simulink model "turbo_controller"  (R2025a)
settings: Solver=FixedStepAuto  StartTime=0.0  StopTime=inf  FixedStep=0.001  RelTol=1e-3
PostLoadFcn:
  | % 自动定位同目录CubeMX文件；不需要外部初始化脚本。
  | codertarget.data.setParameterValue('turbo_controller','STM32CubeMX.ProjectFile',fullfile(fileparts(get_param('turbo_controller','FileName')),'turbo_f407.ioc'));
InitFcn:
  | % 中文说明：按原控制器字段与类型创建三组接口总线；控制参数已内嵌。
  | tc_names=["EValve_Cycle" "EValve_Open" "Eblast_Cycle" "Eblast_Open" "Motor_Cycle" "Motor_Open" "EValve_Enable" "Eblast_Enable" "Motor_Enable" "SWO_Firework" "SWO_BleedAir" "EngineState" "Flag_ECUReset_Clear" "Flag_ECUReset_Save" "Flag_Reset_Enable" "Accelerator" "Nc_dem" "Nc"]; tc_types=["uint16" "uint16" "uint16" "uint16" "uint16" "uint16" "uint8" "uint8" "uint8" "uint8" "uint8" "uint8" "uint8" "uint8" "uint8" "single" "single" "single"];
  | for tc_k=1:numel(tc_names)
  |  tc_e(tc_k)=Simulink.BusElement; tc_e(tc_k).Name=char(tc_names(tc_k)); tc_e(tc_k).DataType=char(tc_types(tc_k));
  | end
  | EngineControl_Out=Simulink.Bus; EngineControl_Out.DataScope='Exported'; EngineControl_Out.Elements=tc_e;
  | clear tc_e tc_names tc_types tc_k
  | tc_names=["savedata1" "savedata2" "savedata3" "savedata4" "savedata5" "savedata6" "savedata7" "savedata8" "savedata9" "savedata10" "savedata11" "savedata12" "savedata13" "savedata14" "savedata15" "savedata16" "savedata17" "savedata18" "savedata19" "savedata20" "savedata21" "savedata22" "savedata23" "savedata24" "savedata25"]; tc_types=["single" "single" "single" "single" "single" "single" "single" "single" "single" "single" "single" "single" "single" "single" "single" "single" "single" "single" "single" "single" "single" "single" "single" "single" "single"];
  | for tc_k=1:numel(tc_names)
  |  tc_e(tc_k)=Simulink.BusElement; tc_e(tc_k).Name=char(tc_names(tc_k)); tc_e(tc_k).DataType=char(tc_types(tc_k));
  | end
  | SaveData_Out=Simulink.Bus; SaveData_Out.DataScope='Exported'; SaveData_Out.Elements=tc_e;
  | clear tc_e tc_names tc_types tc_k
  | tc_names=["senddata1" "senddata2" "senddata3" "senddata4" "senddata5" "senddata6" "senddata7" "senddata8" "senddata9" "senddata10" "senddata11" "senddata12" "senddata13" "senddata14" "senddata15" "senddata16" "senddata17" "senddata18" "senddata19" "senddata20" "senddata21" "senddata22" "senddata23" "senddata24" "senddata25" "senddata26" "senddata27" "senddata28" "senddata29"]; tc_types=["uint8" "uint8" "uint8" "uint8" "uint8" "uint8" "uint8" "uint8" "uint8" "uint8" "uint8" "uint8" "uint8" "uint8" "uint8" "uint8" "uint8" "uint8" "uint8" "uint8" "uint8" "uint8" "uint8" "uint8" "uint8" "uint8" "uint8" "uint8" "uint8"];
  | for tc_k=1:numel(tc_names)
  |  tc_e(tc_k)=Simulink.BusElement; tc_e(tc_k).Name=char(tc_names(tc_k)); tc_e(tc_k).DataType=char(tc_types(tc_k));
  | end
  | SendData_Out=Simulink.Bus; SendData_Out.DataScope='Exported'; SendData_Out.Elements=tc_e;
  | clear tc_e tc_names tc_types tc_k
  | 
  | % 以下为接口中文说明；只设置描述，不改变数值或数据类型。
  | EngineControl_Out.Description='执行控制输出（阀、电机、点火、状态及复位请求）';
  | tc_cn=["EValve_Cycle（主油阀周期计数（每计数2毫秒））" "EValve_Open（主油阀开通计数（每计数2毫秒））" "Eblast_Cycle（副油阀周期计数（每计数2毫秒））" "Eblast_Open（副油阀开通计数（每计数2毫秒））" "Motor_Cycle（起动电机周期计数）" "Motor_Open（起动电机开通计数）" "EValve_Enable（主油阀驱动使能）" "Eblast_Enable（副油阀驱动使能）" "Motor_Enable（起动电机使能）" "SWO_Firework（点火器使能（1开））" "SWO_BleedAir（引气阀使能（1开））" "EngineState（发动机状态）" "Flag_ECUReset_Clear（清除复位恢复状态请求）" "Flag_ECUReset_Save（保存复位恢复数据请求）" "Flag_Reset_Enable（处理器软件复位请求）" "Accelerator（油门／油泵给定控制量）" "Nc_dem（控制目标转速）" "Nc（发动机反馈转速（转每分））"];
  | tc_elements=EngineControl_Out.Elements;
  | for tc_k=1:numel(tc_cn)
  |  tc_elements(tc_k).Description=char(tc_cn(tc_k));
  | end
  | EngineControl_Out.Elements=tc_elements;
  | clear tc_cn tc_elements tc_k
  | SaveData_Out.Description='25项运行记录；字段含义按当前模型数据来源解释';
  | tc_cn=["savedata1（指令回显记录）" "savedata2（入口总温记录（℃））" "savedata3（电源电压记录）" "savedata4（排气温度记录（℃））" "savedata5（标定燃油压力记录）" "savedata6（副油阀占空比记录（％））" "savedata7（主油阀占空比记录（％））" "savedata8（温度修正转速记录）" "savedata9（开关输出及反馈位域）" "savedata10（物理转速记录）" "savedata11（油泵目标给定原始值）" "savedata12（起动电机占空比记录（％））" "savedata13（发动机状态码记录）" "savedata14（故障告警位域记录）" "savedata15（模型记录帧序号）" "savedata16（处理器温度记录（℃））" "savedata17（装订转速记录（沿用旧电源字段名））" "savedata18（导航高度记录）" "savedata19（飞行空速记录）" "savedata20（主阀旧记录位（恒零保留））" "savedata21（第21项保留记录（恒零））" "savedata22（保留记录项22）" "savedata23（保留记录项23）" "savedata24（保留记录项24）" "savedata25（保留记录项25）"];
  | tc_elements=SaveData_Out.Elements;
  | for tc_k=1:numel(tc_cn)
  |  tc_elements(tc_k).Description=char(tc_cn(tc_k));
  | end
  | SaveData_Out.Elements=tc_elements;
  | clear tc_cn tc_elements tc_k
  | SendData_Out.Description='29字段回传及外设命令接口；板端上位机帧只取第3至27字段';
  | tc_cn=["senddata1（回传发送允许标志（不直接上线路））" "senddata2（回传载荷长度25字节）" "senddata3（回传指令回显字节）" "senddata4（总温编码字节（℃＋80））" "senddata5（电源电压编码字节）" "senddata6（排温编码高字节）" "senddata7（排温编码低字节）" "senddata8（燃油压力编码高字节）" "senddata9（燃油压力编码低字节）" "senddata10（副油阀占空比字节（％））" "senddata11（主油阀占空比字节（％））" "senddata12（修正转速编码高字节）" "senddata13（修正转速编码低字节）" "senddata14（驱动及反馈状态位域）" "senddata15（物理转速编码高字节）" "senddata16（物理转速编码低字节）" "senddata17（油泵目标给定高字节（串口二使用））" "senddata18（油泵目标给定低字节（串口二使用））" "senddata19（起动电机占空比命令（串口一使用））" "senddata20（发动机状态码字节）" "senddata21（故障告警位域字节）" "senddata22（帧序号占位（板端另行填写））" "senddata23（处理器温度编码（℃＋50））" "senddata24（控制目标转速编码高字节）" "senddata25（控制目标转速编码低字节）" "senddata26（占位字节（板端改填实测泵速高字节））" "senddata27（占位字节（板端改填实测泵速低字节））" "senddata28（装订转速高字节（本板未发送））" "senddata29（装订转速低字节（本板未发送））"];
  | tc_elements=SendData_Out.Elements;
  | for tc_k=1:numel(tc_cn)
  |  tc_elements(tc_k).Description=char(tc_cn(tc_k));
  | end
  | SendData_Out.Elements=tc_elements;
  | clear tc_cn tc_elements tc_k
  | 
  | 
  | % FRAM模块化事务：接口类型和上电初始状态，随模型保存，无外部初始化文件。
  | clear FM_elements
  | FM_elements(1)=Simulink.BusElement;FM_elements(1).Name='phase';FM_elements(1).DataType='uint8';FM_elements(1).Dimensions=[1 1];FM_elements(1).Description='phase（当前事务阶段）';
  | FM_elements(2)=Simulink.BusElement;FM_elements(2).Name='a';FM_elements(2).DataType='uint8';FM_elements(2).Dimensions=[64 1];FM_elements(2).Description='a（启动时缓存的首区64字节）';
  | FM_elements(3)=Simulink.BusElement;FM_elements(3).Name='active';FM_elements(3).DataType='uint16';FM_elements(3).Dimensions=[1 1];FM_elements(3).Description='active（当前有效记录区地址）';
  | FM_elements(4)=Simulink.BusElement;FM_elements(4).Name='generation';FM_elements(4).DataType='uint32';FM_elements(4).Dimensions=[1 1];FM_elements(4).Description='generation（当前有效记录代号）';
  | FM_elements(5)=Simulink.BusElement;FM_elements(5).Name='record';FM_elements(5).DataType='uint8';FM_elements(5).Dimensions=[64 1];FM_elements(5).Description='record（本次冻结的待写记录）';
  | FM_elements(6)=Simulink.BusElement;FM_elements(6).Name='addr';FM_elements(6).DataType='uint16';FM_elements(6).Dimensions=[1 1];FM_elements(6).Description='addr（本次备用写入地址）';
  | FM_elements(7)=Simulink.BusElement;FM_elements(7).Name='lastSave';FM_elements(7).DataType='single';FM_elements(7).Dimensions=[1 1];FM_elements(7).Description='lastSave（上次开始保存的秒数）';
  | FM_elements(8)=Simulink.BusElement;FM_elements(8).Name='lastState';FM_elements(8).DataType='uint8';FM_elements(8).Dimensions=[1 1];FM_elements(8).Description='lastState（上次保存时的发动机状态）';
  | FM_elements(9)=Simulink.BusElement;FM_elements(9).Name='boot';FM_elements(9).DataType='boolean';FM_elements(9).Dimensions=[1 1];FM_elements(9).Description='boot（启动记录是否允许恢复）';
  | FM_elements(10)=Simulink.BusElement;FM_elements(10).Name='consumed';FM_elements(10).DataType='boolean';FM_elements(10).Dimensions=[1 1];FM_elements(10).Description='consumed（本次启动恢复通知是否已发送）';
  | FM_elements(11)=Simulink.BusElement;FM_elements(11).Name='payload';FM_elements(11).DataType='uint8';FM_elements(11).Dimensions=[20 1];FM_elements(11).Description='payload（当前20字节恢复内容）';
  | ... (+35 lines)
model workspace (MAT data in the model file):
  CRC16_Table_Reference = [0 4129 8258 12387 16516 20645 24774 28903 33032 37161 41290 45419 ... (256 elements, 256x1)]
  PE_Kaer = [0.15402 0.15402 0.12264 0.10076 0.09481 0.07601 0.07111 0.0569 0.05198 0.04926 0.05308 0.04325 ... (13 elements, 1x13)]
  PE_Nr = [21.2982 61.4260372 67.7475458 72.7394382 76.845934 80.6988798 83.8449282 86.6491912 88.9382406 89.178606 91.1938214 93.4068058 ... (13 elements, 1x13)]
  PE_Pump_Translate = 33.5999984741
  PE_RotaSpeed_Translate = 860
  PE_Taer = [0.4939154 0.4939154 0.40780982 0.34066978 0.31622756 0.30405716 0.34300244 0.26785022 0.37393554 0.23914836 0.44563948 0.31044662 ... (13 elements, 1x13)]
  PF_ACCFULLRANGE = 3360
  PF_Flag_ECUReset = 0
  PF_Flag_rx_suc = 1
  PF_Gear_Info = [40000; 45000; 50000; 55000; 57000; 59000; 60000; 61000; 61000; 61000; 61000; 61000]
  PF_K_TiaoJie = 1
  PF_Kpu = 10
  PF_MySet_Rxdata = [0 0 0 0 0 0 0 0 0 0 0 0 ... (50 elements, 50x1)]
  PF_MyUsart1_Rxdata = [0 0 0 0 0 0 0 0 0 0 0 0 ... (50 elements, 50x1)]
  PF_MyUsart2_Rxdata = [0 0 0 0 0 0 0 0 0 0 0 0 ... (50 elements, 50x1)]
  PF_Reset_Information = [0 0 0 0 0 0 0 0 0 0 0 0 ... (20 elements, 20x1)]
  PF_Sensor_X1_T4 = [0 4095]
  PF_Sensor_X2_T4 = [0 1.66666698456]
  PF_Sensor_X3_T4 = [0 504 999 1497 2010 2529 3051 3568 4076 4571 4959]
  PF_Sensor_X_P2 = [0.5 3]
  PF_Sensor_X_Poil = [0.5 3]
  PF_Sensor_X_T1t = [-50 300]
  PF_Sensor_X_Vpower = [0 3]
  PF_Sensor_X_Vpump = [0 3]
  PF_Sensor_Y1_T4 = [0 3]
  PF_Sensor_Y2_T4 = [0 5000]
  PF_Sensor_Y3_T4 = [0 100 200 300 400 500 600 700 800 900 980]
  PF_Sensor_Y_P2 = [0 1000]
  PF_Sensor_Y_Poil = [0 1000]
  PF_Sensor_Y_T1t = [-50 300]
  PF_Sensor_Y_Vpower = [0 33]
  PF_Sensor_Y_Vpump = [0 33]
  PG_CtrlMode_CloseLoop : mpt.Parameter (value not decoded)
  PG_CtrlMode_ManualAcc : mpt.Parameter (value not decoded)
  PG_CtrlMode_Origin : mpt.Parameter (value not decoded)
  PG_CtrlMode_Start : mpt.Parameter (value not decoded)
  PG_CtrlMode_Stop : mpt.Parameter (value not decoded)
  PG_ES_Clp : mpt.Parameter (value not decoded)
  PG_ES_EngStart : mpt.Parameter (value not decoded)
  PG_ES_Manual : mpt.Parameter (value not decoded)
  PG_ES_Origin : mpt.Parameter (value not decoded)
  PG_ES_Stop : mpt.Parameter (value not decoded)
  PG_Instr_BleedAirSet : mpt.Parameter (value not decoded)
  PG_Instr_CloseLoop : mpt.Parameter (value not decoded)
  PG_Instr_ECUReSet : mpt.Parameter (value not decoded)
  PG_Instr_EValveSet : mpt.Parameter (value not decoded)
  PG_Instr_EblastSet : mpt.Parameter (value not decoded)
  PG_Instr_Erase : mpt.Parameter (value not decoded)
  PG_Instr_FireWorkSet : mpt.Parameter (value not decoded)
  PG_Instr_ManualPlus : mpt.Parameter (value not decoded)
  PG_Instr_ManualrReduce : mpt.Parameter (value not decoded)
  PG_Instr_MotorSet : mpt.Parameter (value not decoded)
  PG_Instr_OilSet : mpt.Parameter (value not decoded)
  PG_Instr_SelfCheck : mpt.Parameter (value not decoded)
  PG_Instr_Start : mpt.Parameter (value not decoded)
  PG_Instr_Stop : mpt.Parameter (value not decoded)
  PG_Instr_StopZero : Simulink.Parameter (value not decoded)
  PG_Location_Air : Simulink.Parameter (value not decoded)
  PG_Location_Gnd : Simulink.Parameter (value not decoded)
  PG_ServoCtrlMode_CloseLoop : Simulink.Parameter (value not decoded)
  PG_ServoCtrlMode_CloseLoopMax : Simulink.Parameter (value not decoded)
  PG_ServoCtrlMode_CloseLoopMin : Simulink.Parameter (value not decoded)
  PG_ServoCtrlMode_ManualAcc : Simulink.Parameter (value not decoded)
  PG_ServoCtrlMode_ManualAccMax : Simulink.Parameter (value not decoded)
  PG_ServoCtrlMode_ManualAccMin : Simulink.Parameter (value not decoded)
  PG_SpeedDot_Permit : Simulink.Parameter (value not decoded)
  PL_EngineModel_Actuator = [0 10 100]
  PL_EngineModel_EngineStar_Press_P2 = [1013 1098.4 1099.144828 1099.931034 1103.613793 1162.662069 1143.793103 1131.006897 1123.186207 1117.6 1114 1111.806897 ... (127 elements, 1x127)]
  PL_EngineModel_EngineStar_RotaSpeed = [200 2000 9584 9660 10220 10240 10260 10288 10308 10368 10380 10408 ... (127 elements, 1x127)]
  PL_EngineModel_EngineStar_Temp_Exhaust = [128 129 129.1 130 131 131.1 132 133 134 134.1 135 135.1 ... (127 elements, 1x127)]
  PL_EngineModel_EngineStar_Time = [0.05 0.1 0.15 0.2 0.25 0.3 0.35 0.4 0.45 0.5 0.55 0.6 ... (127 elements, 1x127)]
  PL_EngineModel_IdleAbove_Nr = [0 21.2982 61.4260372 67.7475458 72.7394382 76.845934 80.6988798 83.8449282 86.6491912 88.9382406 89.178606 91.1938214 ... (14 elements, 1x14)]
  PL_EngineModel_IdleAbove_P2r = [0.986923266716 1.57907722675 1.81593881076 1.99358499877 2.23044658278 2.43770046879 2.65482358747 2.84233900814 3.03972366149 3.18776215149 3.25684678016 3.3950160375 ... (14 elements, 1x14)]
  PL_EngineModel_IdleAbove_Tempr = [0.0536001429337 1.07200285867 1.63301768805 1.63659103091 1.66875111667 1.72592460247 1.77595140254 1.86171163123 1.95461854565 2.03323208862 2.03323208862 2.13685903162 ... (14 elements, 1x14)]
  PL_EngineModel_IdleAbove_Ter = [0.42434128 0.42434128 0.42434128 0.30669408 0.23570008 0.22150128 0.1997974 0.23803274 0.16115638 0.24279948 0.13600422 0.31308354 ... (14 elements, 1x14)]
  PL_EngineModel_IdleAbove_Wfr = [0 10.142 23.8337 27.8905 31.9473 36.0041 40.0609 44.1177 48.1745 52.2313 52.7384 56.7952 ... (14 elements, 1x14)]
  PL_EngineModel_Press_P2 = [400 400 400 400 400 400 400 400 400 400]
  PL_EngineModel_Rotaspeed = [0 20000 96400]
  PL_EngineModel_Temp_Exhaust = [500 500 500 500 500 500 500 500 500 500]
  PL_Kaer = [0.1 0.1 0.1 0.1 0.1 0.1]
  PL_Nr = [50 60 70 80 90 100]
  PL_Taer = [0.1 0.1 0.1 0.1 0.1 0.1]
  Sig : Simulink.Signal (value not decoded)
  Ts_ms : Simulink.Parameter (value not decoded)
  false : Simulink.Parameter (value not decoded)
  true : Simulink.Parameter (value not decoded)
symbols that are objects in the model workspace (value not decoded): PG_CtrlMode_CloseLoop, PG_CtrlMode_ManualAcc, PG_CtrlMode_Origin, PG_CtrlMode_Start, PG_CtrlMode_Stop, PG_ES_Clp, PG_ES_EngStart, PG_ES_Manual, PG_ES_Origin, PG_ES_Stop, PG_Instr_BleedAirSet, PG_Instr_CloseLoop, PG_Instr_EblastSet, PG_Instr_ECUReSet, PG_Instr_Erase, PG_Instr_EValveSet, PG_Instr_FireWorkSet, PG_Instr_ManualPlus, PG_Instr_ManualrReduce, PG_Instr_MotorSet, PG_Instr_OilSet, PG_Instr_SelfCheck, PG_Instr_Start, PG_Instr_Stop, PG_Instr_StopZero, PG_ServoCtrlMode_CloseLoop, PG_ServoCtrlMode_CloseLoopMax, PG_ServoCtrlMode_CloseLoopMin, PG_ServoCtrlMode_ManualAcc, PG_ServoCtrlMode_ManualAccMax, PG_ServoCtrlMode_ManualAccMin, Ts_ms
libraries: simulink x97, stm32blockslib x10, stm32f4xxblockslib x8
(part 2 of 26)

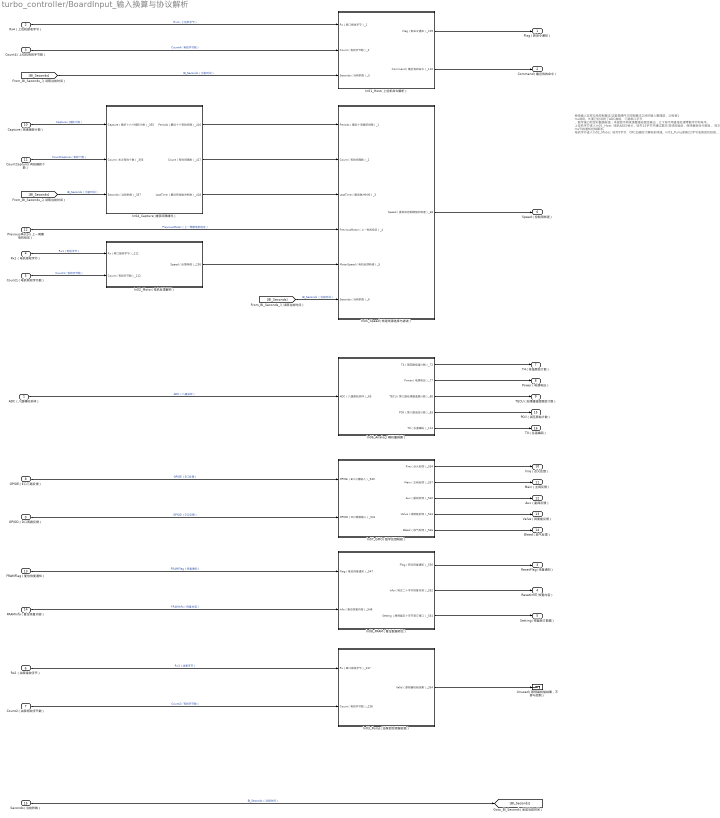
== system turbo_controller/BoardInput_输入换算与协议解析 ==
  note: 板级输入怎样交给控制算法
      |
      | 这里是硬件与控制算法之间的输入整理层，父级每1 ms调用。外面已经读到了ADC数组、三路串口字节
      | 、数字端口和定时器捕获值；本层把不同来源整理成固定输出，让下游不用直接处理零散字节和电平。
      |
      | 上位机字节进入In01_Host，找到AA55帧头，收齐14字节并通过累加/异或校验后，保持最新命令数组，
      | 按20 ms节拍通知控制算法。
      | 电机字节进入In02_Motor，收齐9字节、CRC正确后计算电机转速。In03_Pump保留22字节油泵回包校验
      | ，但这个输入侧预留结果不参与实际泵速回传；实际泵反馈处理在BoardOutput/Out01_Pump。
      |
      | 定时器数据先到In04_Capture，用相邻计数差建立最近10项间隔缓存；再到In05_Speed，以电机反馈和
      | 捕获估算两种来源选出控制转速。控制转速每20 ms更新，其余毫秒保持。
      |
      | ADC数据进入In06_Analog：第1项换电源电压，第3、4、8项转交芯片温度/排温/油压计数，第5和7项一
      | 起反算总温，第2和6项暂未使用。
      | GPIOE/GPIOD进入In07_GPIO，按硬件电平极性映射成五个反馈；FRAM通知和20字节内容由In08_FRAM转
      | 交。
      |
      | 输出再经过根层ControlRate送入COMMRead_ISM。注意本层多数温度和油压仍是原始计数，下游ISM才做
      | 标定滤波；父级1 ms调用不等于所有传感器每1 ms获得新采样。
  ADC（八路模拟采样） : Inport
  Rx4（上位机接收字节） : Inport  Port=2
  Count4（上位机有效字节数） : Inport  Port=3
  Rx1（电机接收字节） : Inport  Port=4
  Count1（电机有效字节数） : Inport  Port=5
  Rx2（油泵接收字节） : Inport  Port=6
  Count2（油泵有效字节数） : Inport  Port=7
  GPIOE（E口三路反馈） : Inport  Port=8
  GPIOD（D口两路反馈） : Inport  Port=9
  Capture（转速捕获计数） : Inport  Port=10
  CountCapture（有效捕获个数） : Inport  Port=11
  PreviousMotor（上一周期电机给定） : Inport  Port=12
  FRAMFlag（复位恢复通知） : Inport  Port=13
  FRAMInfo（复位恢复内容） : Inport  Port=14
  Seconds（当前秒数） : Inport  Port=15
  In01_Host（上位机命令解析） : Subsystem  Description=|  TreatAsAtomicUnit=on
      | 从上位机字节流中取出一条可靠命令
      | 
      | 串口每次提供一个字节数组和实际接收数量。数组容量不是有效数据长度，必须只处理本次计数范围内的字节；否则尾部旧数据可能被误当作新命令。
      | 
      | Receive按字节顺序调用Collect：先找十六进制AA、55两个帧头，再把后续数据放入14字节缓存。收齐后交Verify检查累加校验和异或校验。两种校验都一致才接收这帧，失败时不覆盖上次有效命令。
      | 
      | 通过的14字节放进原控制算法沿用的50项接口，未用部分补零，并保存“有新命令”等待通知。每20 ms节拍把这次新命令标志交给根层ControlRate；没有新有效帧时仍保留上次内容，但不应把保持内容解释成又收到一条命令。
      | 
      | 输出的命令数组随后进入COMMRead_ISM/CMMRead。那里的Instr_Analyse才把FC等原始命令字节解释成内部Instr，SpeedLoad_Analyse解析目标转速。因此本层负责可靠收帧，尚未决定发动机该启动还是停车。
  In02_Motor（电机反馈解析） : Subsystem  Description=|  TreatAsAtomicUnit=on
      | 电机反馈字节怎样变成转速
      | 
      | 输入来自USART1电机串口，包括字节数组和实际有效数量。逐字节识别AA55帧头、收齐9字节后，先核对CRC16；只有本次新帧通过校验，才采用第6、7字节。
      | 
      | 第6项为高字节，第7项为低字节，先合成16位原始数：
      | 原始数 = 第6字节 × 256 + 第7字节；
      | 电机反馈转速 = floor(原始数 / 3)。
      | 例如高字节1、低字节44合成300，除以3后得到100。除3是本工程保留的反馈比例，floor表示向下取整。
      | 
      | 通过校验后更新并记住转速；没有新完整帧或CRC失败时保持上次有效反馈。保持旧值不代表电机这一毫秒又发来了同样的数据。
      | 
      | 结果作为In05_Speed的一种转速来源。上一电机给定非零时，它的优先级高于定时器捕获估算。该模块是接收解析，不负责发电机控制命令。
  In03_Pump（油泵回包预留校验） : Subsystem  Description=|  TreatAsAtomicUnit=on
      | 输入侧油泵回包的预留检查
      | 
      | 本模块接收油泵串口字节和有效数量，内部Receive按AA55帧头拼接22字节帧，再检查CRC16。分批到达的帧可以依靠缓存接着收，校验失败不会变成有效帧。
      | 
      | 它保留的是输入侧原有预留校验路径，当前该结果没有用来更新控制转速或实际回传泵速。不要因为这里名为Pump，就把它当成最终泵速反馈来源。
      | 
      | 实际用于上位机回传的油泵反馈，在BoardOutput/Out01_Pump中处理：同样检查22字节帧，提取第6、7字节并作0.875/0.125平滑。本模块没有取代那条路径，也不生成发往油泵的控制命令。
  In04_Capture（捕获间隔缓存） : Subsystem  Description=|  TreatAsAtomicUnit=on
      | 捕获间隔缓存：把脉冲发生时刻整理成最近十个时间间隔
      | 
      | 输入Capture是TIM3本批捕获读数，最多16项；输入Count只说明本批有几项新读数，Seconds为本次处理时刻，单位秒。当前定时器每增加1计数相当于1微秒。
      | 
      | 按四块阅读：
      | Step01逐项取出本批有效捕获，超过本批数量或第16项就结束循环；
      | Step02保存上次捕获、十项间隔、写入位置、累计有效数和最近有效时间；
      | Step03根据本项捕获计算间隔，决定是否更新缓存和状态；
      | Step04只整理三个输出的维度，送后续测速。
      | 
      | Step02与Step03之间是状态反馈，不是先等一个额外毫秒再处理。Loop会在同一次调用内遍历本批多个捕获；一个批次的末项读数也会留作下一批首项的差分基准。
      | 
      | 输出Periods为最近十个间隔，Count为缓存里真正有效的间隔个数，LastTime为最近接受正间隔的处理时刻。输出Count与输入Count不是同一个数量。这里不直接输出转速；去极值与每转3脉冲换算在In05_Speed/CaptureSpeed完成。
  In05_Speed（转速来源选择与滤波） : Subsystem  Description=|  TreatAsAtomicUnit=on
      | 电机反馈与捕获估速怎样选成控制转速
      | 
      | 这里有两种候选转速：电机串口反馈Motor，以及十项捕获间隔算出的Captured。输出Speed送根层ControlRate，再到ISM作进一步异常判断和滤波。
      | 
      | 先由Clock20ms产生每20 ms更新许可。CaptureSpeed从有效间隔中去掉一个最大和一个最小，估算转速，并给出分母有效标志。Status判断：上一电机给定是否非零、是否还在10次节拍等待中、脉冲是否超过0.1 s未更新、间隔是否至少3项。
      | 
      | Select按顺序选择：电机给定非零时优先Motor，并把等待计数清零；退出电机后先保持旧Speed，等待10次20 ms节拍，约0.2 s后再尝试捕获估速。
      | 等待结束后，脉冲超时则给零；未超时且数量足够、分母有效才采用Captured，否则保持旧值。
      | 
      | 非20 ms更新时刻，Speed和等待计数都保持。因此“父级每1 ms运行”并不是每1 ms都切换转速来源。Held是上次控制转速，WaitCount是切换过程的记忆。
  In06_Analog（模拟量换算） : Subsystem  Description=|  TreatAsAtomicUnit=on
      | 八路ADC怎样变成五类测量数据
      | 
      | 这里收到的是ADC1每20毫秒采集的一组八项计数，数值约为0～4095。计数表示输入电压在量程中的位置，还不能直接当成摄氏度或油压。本层先按数组位置分开处理，再把五类结果交给根层ControlRate，进入COMMRead_ISM/ISM继续标定。
      | 
      | 1 电源电压取第1项。先转成single以便做小数运算，再计算：
      | 电源电压 = 第1项计数 × 48 / 4096，单位V。
      | 例如计数2048对应24 V。这里已完成电源电压换算，ISM随后直接把它放入Sensor.Vpower，用于22 V欠压判断、记录和回传。
      | 
      | 2 控制器温度取第3项。这是芯片内部温度传感器的计数。本层只转成single后输出TECU；下一级Calibrating_Tecu才把它换成电压和摄氏温度。本层没有把它当成温度直接使用。
      | 
      | 3 排温取第4项，油压取第8项。两路在这里均只转成single，分别输出T4和POil。后面的Calibrating_T4用三级查表得到排温，Calibrating_Poil用两级查表得到油压，然后各自低通滤波。它们离开本层时仍是ADC计数。
      | 
      | 4 总温需要第5和第7两项一起计算。第5项提供参考电压，第7项提供传感器电压；TotalTemperature先反算电阻，再换算温度，最后加80形成T0编码。例如计算温度25 ℃时，编码为105；后面的Calibrating_T0再减80。
      | 
      | 5 第2、第6项当前没有取出参与运算。Format/Reshape只整理输出的数组形状，不改变数值；single转换也不是物理标定。
      | 
      | 因此，五个输出不能按同一种单位解释：Power是V，T4/TECU/POil仍是计数，T0是带80偏置的温度编码。这里的“数组第1项”对应硬件ADC通道2，并不是硬件通道1。
  In07_GPIO（数字反馈映射） : Subsystem  Description=|  TreatAsAtomicUnit=on
      | 把五路硬件电平解释成控制反馈
      | 
      | 输入GPIOE按根层顺序包含PE13、PE14、PE15；GPIOD包含PD8、PD9。Selector按数组位置取出，再经过原有极性映射、single转换和形状整理，形成Fire、Main、Aux、Valve、Bleed五个输出。
      | 
      | E口三项分别提供主阀、副阀、引气阀相关反馈；D口两项提供点火与阀使能/告警相关反馈。逻辑有效方向要结合本页取反支路：硬件低电平不一定表示软件“无告警”，因此不能把原始0/1直接当动作状态。
      | 
      | 本层只整理反馈，不生成阀门驱动。输出经ControlRate进入ISM，按SWI_Firework、SWI_EValve等名称进入Sensor总线，供记录回传和有关检查使用。Format/Reshape只调整形状，类型转换不改变电路有效极性。
  In08_FRAM（复位数据转交） : Subsystem  Description=|  TreatAsAtomicUnit=on
      | 把FRAM恢复结果交到旧控制接口
      | 
      | 输入是FRAM事务模块给出的一次性恢复通知和20字节恢复内容。本层保持原有接口的数据类型和维度，将两者转交为ResetFlag与ResetInfo，供根层20 ms控制交接。
      | 
      | 这里不读取SPI，不重算CRC，也不从20字节中提取油泵给定或转速。SPI收发、双区校验和一次性通知在FRAM_复位恢复事务中完成；字段解码在COMMRead_ISM/ECUReset_Information_Read完成。
      | 
      | 通知表示“现在允许考虑恢复这份内容”，数据数组表示“要恢复什么”，二者不能分开理解。数组有数值本身不代表恢复已启用。
      | 
      | 当前COMMRead_ISM内部把实际恢复解码许可接到false常量，外部ResetFlag被终止。因此本模块具备通知和内容的转交，但现有后级连线没有真正采用这一路恢复许可。
  Unused（原预留校验结果，不参与控制） : Terminator
  Flag（新命令通知） : Outport
  Command（最近有效命令） : Outport  Port=2
  ResetFlag（恢复通知） : Outport  Port=3
  ResetInfo（恢复内容） : Outport  Port=4
  Setting（预留装订数据） : Outport  Port=5
  Speed（控制用转速） : Outport  Port=6
  T4（排温原始计数） : Outport  Port=7
  Power（电源电压） : Outport  Port=8
  TECU（处理器温度原始计数） : Outport  Port=9
  Fire（点火反馈） : Outport  Port=10
  Main（主阀反馈） : Outport  Port=11
  Aux（副阀反馈） : Outport  Port=12
  Valve（阀使能反馈） : Outport  Port=13
  Bleed（放气反馈） : Outport  Port=14
  POil（油压原始计数） : Outport  Port=15
  T0（总温编码） : Outport  Port=16
  wires:
  Seconds（当前秒数）/1 -> [BI_Seconds]  "BI_Seconds（当前时间）"
  In01_Host（上位机命令解析）/2(Command（最近有效命令）_110) -> Command（最近有效命令）/1
  In01_Host（上位机命令解析）/1(Flag（新命令通知）_109) -> Flag（新命令通知）/1
  [BI_Seconds] -> In01_Host（上位机命令解析）/3(Seconds（当前秒数）_3)  "BI_Seconds（当前时间）"
  Count4（上位机有效字节数）/1 -> In01_Host（上位机命令解析）/2(Count（有效字节数）_2)  "Count4（有效字节数）"
  Rx4（上位机接收字节）/1 -> In01_Host（上位机命令解析）/1(Rx（串口接收字节）_1)  "Rx4（上位机字节）"
  In03_Pump（油泵回包预留校验）/1(Valid（原预留校验结果）_354) -> Unused（原预留校验结果，不参与控制）/1
  Count2（油泵有效字节数）/1 -> In03_Pump（油泵回包预留校验）/2(Count（有效字节数）_238)  "Count2（有效字节数）"
  Rx2（油泵接收字节）/1 -> In03_Pump（油泵回包预留校验）/1(Rx（串口接收字节）_237)  "Rx2（油泵字节）"
  In07_GPIO（数字反馈映射）/5(Bleed（放气反馈）_546) -> Bleed（放气反馈）/1
  In07_GPIO（数字反馈映射）/4(Valve（阀使能反馈）_543) -> Valve（阀使能反馈）/1
  In07_GPIO（数字反馈映射）/3(Aux（副阀反馈）_540) -> Aux（副阀反馈）/1
  In07_GPIO（数字反馈映射）/2(Main（主阀反馈）_537) -> Main（主阀反馈）/1
  In07_GPIO（数字反馈映射）/1(Fire（点火反馈）_534) -> Fire（点火反馈）/1
  GPIOD（D口两路反馈）/1 -> In07_GPIO（数字反馈映射）/2(GPIOD（D口两路输入）_531)  "GPIOD（D口反馈）"
  GPIOE（E口三路反馈）/1 -> In07_GPIO（数字反馈映射）/1(GPIOE（E口三路输入）_530)  "GPIOE（E口反馈）"
  In08_FRAM（复位数据转交）/3(Setting（原预留五十字节装订接口）_554) -> Setting（预留装订数据）/1
  In08_FRAM（复位数据转交）/2(Info（转交二十字节恢复内容）_552) -> ResetInfo（恢复内容）/1
  In08_FRAM（复位数据转交）/1(Flag（转交恢复通知）_550) -> ResetFlag（恢复通知）/1
  FRAMInfo（复位恢复内容）/1 -> In08_FRAM（复位数据转交）/2(Info（复位恢复内容）_548)  "FRAMInfo（恢复内容）"
  FRAMFlag（复位恢复通知）/1 -> In08_FRAM（复位数据转交）/1(Flag（复位恢复通知）_547)  "FRAMFlag（恢复通知）"
  In05_Speed（转速来源选择与滤波）/1(Speed（提供给控制模型的转速）_68) -> Speed（控制用转速）/1
  [BI_Seconds] -> In05_Speed（转速来源选择与滤波）/6(Seconds（当前秒数）_6)  "BI_Seconds（当前时间）"
  In02_Motor（电机反馈解析）/1(Speed（反馈转速）_236) -> In05_Speed（转速来源选择与滤波）/5(MotorSpeed（电机反馈转速）_5)
  PreviousMotor（上一周期电机给定）/1 -> In05_Speed（转速来源选择与滤波）/4(PreviousMotor（上一电机给定）_4)  "PreviousMotor（上一周期电机给定）"
  In04_Capture（捕获间隔缓存）/3(LastTime（最近有效脉冲秒数）_418) -> In05_Speed（转速来源选择与滤波）/3(LastTime（最近脉冲时间）_3)
  In04_Capture（捕获间隔缓存）/2(Count（有效间隔数）_417) -> In05_Speed（转速来源选择与滤波）/2(Count（有效间隔数）_2)
  In04_Capture（捕获间隔缓存）/1(Periods（最近十个有效间隔）_416) -> In05_Speed（转速来源选择与滤波）/1(Periods（最近十项捕获间隔）_1)
  Count1（电机有效字节数）/1 -> In02_Motor（电机反馈解析）/2(Count（有效字节数）_112)  "Count1（有效字节数）"
  Rx1（电机接收字节）/1 -> In02_Motor（电机反馈解析）/1(Rx（串口接收字节）_111)  "Rx1（电机字节）"
  [BI_Seconds] -> In04_Capture（捕获间隔缓存）/3(Seconds（当前秒数）_357)  "BI_Seconds（当前时间）"
  CountCapture（有效捕获个数）/1 -> In04_Capture（捕获间隔缓存）/2(Count（本次有效个数）_356)  "CountCapture（有效个数）"
  Capture（转速捕获计数）/1 -> In04_Capture（捕获间隔缓存）/1(Capture（最多十六个捕获计数）_355)  "Capture（捕获计数）"
  In06_Analog（模拟量换算）/5(T0（总温编码）_113) -> T0（总温编码）/1
  In06_Analog（模拟量换算）/4(POil（第八路油压计数）_83) -> POil（油压原始计数）/1
  In06_Analog（模拟量换算）/3(TECU（第三路处理器温度计数）_80) -> TECU（处理器温度原始计数）/1
  In06_Analog（模拟量换算）/2(Power（电源电压）_77) -> Power（电源电压）/1
  In06_Analog（模拟量换算）/1(T4（第四路排温计数）_72) -> T4（排温原始计数）/1
  ADC（八路模拟采样）/1 -> In06_Analog（模拟量换算）/1(ADC（八路原始采样）_69)  "ADC（八路采样）"

== system turbo_controller/BoardOutput_串口封装与阀门时序 ==
  note: 控制要求怎样变成板上的电平与串口帧
      |
      | 上层ControlOut给出油泵、电机、阀门、点火等要求，SendData给出回传协议字段。本层按1 ms任务运
      | 行，把这些要求变成外层STM32驱动块能直接接收的数据，而不是重新决定发动机处于哪种控制模式。
      |
      | Out01_Pump接收油泵串口回包，校验22字节帧并平滑泵速，用于回传。
      | Out02_Timing把主副阀的周期与开通计数变成开关节奏，再按电路低有效极性形成GPIOE/GPIOD输出；
      | 点火请求形成9 ms开、1 ms关的循环。
      |
      | Out03_Telemetry按20 ms节拍，将回传字段、帧号和实际泵速排成28字节内容，再追加两项校验，形成
      | 30字节上位机帧。
      | Out04_Command按20 ms节拍生成两路9字节外设帧。电机命令高字节固定0，油泵命令使用原高低给定字
      | 节，CRC只覆盖两个命令字节。
      |
      | Out05_Handoff集中转交电平、三路串口帧和有效长度，并处理软件复位请求。实际UART/GPIO动作发生
      | 在根层官方硬件块中；生成一帧数据不等于串口已经物理发送完成。
  Control（执行控制总线） : Inport
  Send（回传及外设命令总线） : Inport  Port=2
  PumpRx（油泵反馈字节） : Inport  Port=3
  PumpCount（油泵有效字节数） : Inport  Port=4
  Seconds（当前秒数） : Inport  Port=5
  Out01_Pump（泵反馈解析与滤波） : Subsystem  Description=|  TreatAsAtomicUnit=on
      | 油泵反馈怎样解析并平滑
      | 
      | 这里接收USART2的油泵回包字节和有效数量。逐字节寻找AA55帧头，收齐22字节并通过CRC16后，才取第6、7字节，按高字节在前合成原始泵速：
      | 本次原始反馈 = 高字节 × 256 + 低字节。
      | 
      | 有效新帧到来时，不立即把输出完全跳到新值，而按原模型加权：
      | 本次泵速 = 0.875 × 上次泵速 + 0.125 × 本次原始反馈。
      | 例如上次输出800、新反馈1000，本次输出825。后续继续收到1000时再逐步接近，减少反馈跳动。
      | 
      | 没有新有效帧时保持旧输出。这里的0.125更新只随有效回包发生，不能当成每毫秒都用相同数据再滤波一次。
      | 
      | 该反馈交给Out03_Telemetry，拆成高低字节填入上位机回传帧；它不决定油泵的给定值。输入侧In03_Pump是另一条预留校验路径，不能与本模块混淆。
  Out02_Timing（阀门与点火时序） : Subsystem  Description=|  TreatAsAtomicUnit=on
      | 阀门周期和点火请求怎样变成引脚电平
      | 
      | 输入来自执行控制总线，本层每1 ms运行。先取出主阀、副阀的Enable、Cycle、Open，以及点火与引气请求。Cycle/Open是周期内的计数，不是已经生成的电平。
      | 
      | 主阀和副阀分别交给MainValve、AuxValve。两者按2 ms节拍推进周期位置，位置小于Open时逻辑开启；使能为零或Cycle为零时关闭。例：Cycle=30、Open=15，对应约60 ms周期、前30 ms开启。
      | Ignition把非零点火请求变成10 ms循环中的前9 ms接通、最后1 ms断开。
      | 
      | 然后才做电路极性映射：主阀、副阀、引气和点火的实际驱动支路按本页取反/比较变成低有效电平。软件On=true表示要求开启，不意味着GPIO一定为高。
      | 
      | PortE顺序为副阀、主阀、引气的低有效电平，对应根层PE7、PE8、PE10。
      | PortD顺序为主阀使能高有效镜像、主阀逻辑开启镜像、点火低有效电平，对应PD11、PD12、PD13。
      | 
      | 输出只整理为三项数组交给官方Digital Port Write。模式选择已经在CLM完成，本层按收到的要求排时序。
  Out03_Telemetry（上位机回传组帧） : Subsystem  Description=|  TreatAsAtomicUnit=on
      | 把回传字段组成一帧上位机数据
      | 
      | 上层Send总线是若干字段，不是可以直接发出的最终串口字节数组。本模块同时接收Out01_Pump解析出的实际泵速，并按Clock20ms的许可，每20 ms生成一次通信更新。
      | 
      | FrameCounter在更新时推进0～255循环帧号；PumpBytes把平滑泵速取整为16位，再拆成高、低两字节。
      | Payload先按原协议映射字段，加入AA55及类型01头部，然后明确覆盖第23字节帧号、第27字节泵速高字节、第28字节泵速低字节。
      | 
      | Checksum对这28字节计算累加和异或校验，并追加到末尾，形成30字节帧。发送长度与回传开关、更新节拍共同决定本周期是否交给UART4发送，非更新时不能把相同数组误当新帧不断发送。
      | 
      | 外层Bus Creator3有29个字段，那是总线接口数量；这里的30是最终串口帧字节数，二者不应直接比较成“长度不一致”。实际硬件发送由根层UART4_发送协议帧完成。
  Out04_Command（电机及油泵指令） : Subsystem  Description=|  TreatAsAtomicUnit=on
      | 给电机和油泵各生成一帧控制命令
      | 
      | 这里使用上层执行控制和回传字段，按20 ms节拍生成两路外设命令，而不是解析外设回包。两路协议均为9字节：
      | AA 55 03 00 02 命令高字节 命令低字节 CRC高字节 CRC低字节。
      | 
      | 电机这一路把命令高字节固定为0，低字节采用原电机给定。油泵这一路采用原有油泵给定的高低两个字节；不能把两路的字节来源互换。
      | MotorFrame和PumpFrame各自只对两个命令字节计算CRC，不把前五项固定头部加入校验。
      | 
      | 到20 ms更新且相应发送条件成立时，输出帧和有效长度交Out05_Handoff，再送根层USART1/USART2发送模块。数据值为0也可能是一条有意义的停机命令，因此发送许可和命令是否为0是不同判断。
  Out05_Handoff（输出交接与软件复位） : Subsystem  Description=|  TreatAsAtomicUnit=on
      | 把准备好的输出交给硬件并处理复位请求
      | 
      | 上游已经完成电平时序、上位机帧、电机帧和油泵帧。本层把这些结果按固定字段组成交接总线，转回根层GPIO与UART模块所需的端口，不在这里重新计算温压或改变控制模式。
      | 
      | 串口的数据数组和有效长度必须配套：长度为0表示本周期不发送，命令内容为0却可能是有效的停泵/停电机帧，不能据数值0丢弃。
      | 
      | 另一支取出Flag_Reset_Enable，与0比较后转成复位服务的0/1执行许可。ResetService只在请求有效时执行目标端软件复位；正常电脑仿真走空实现。
      | 
      | 输入依赖使复位处理与本周期输出计算有明确交接关系，但它没有等待硬件UART发送完成的反馈。因此不能把这里解释为已经确认所有字节发完才复位。
  Outputs（拆出原有八项输出） : BusSelector  OutputSignals=portE,portD,tx4,len4,tx1,len1,tx2,len2
  PortE（E口三路电平） : Outport
  PortD（D口三路电平） : Outport  Port=2
  Tx4（上位机回传帧） : Outport  Port=3
  Length4（回传发送长度） : Outport  Port=4
  Tx1（电机指令帧） : Outport  Port=5
  Length1（电机发送长度） : Outport  Port=6
  Tx2（油泵指令帧） : Outport  Port=7
  Length2（油泵发送长度） : Outport  Port=8
  wires:
  Seconds（当前秒数）/1 -> [BO_Seconds]  "BO_Seconds（当前时间）"
  Send（回传及外设命令总线）/1 -> [BO_Send]  "BO_Send（回传命令）"
  Control（执行控制总线）/1 -> [BO_Control]  "BO_Control（执行控制）"
  Out05_Handoff（输出交接与软件复位）/1(Output（完整板级输出总线）_996) -> Outputs（拆出原有八项输出）/1
  Out04_Command（电机及油泵指令）/4(Length2（油泵发送长度）_985) -> Out05_Handoff（输出交接与软件复位）/9(len2（油泵发送长度）_994)
  Out04_Command（电机及油泵指令）/3(Tx2（油泵九字节指令）_984) -> Out05_Handoff（输出交接与软件复位）/8(tx2（油泵指令帧）_993)
  Out04_Command（电机及油泵指令）/2(Length1（电机发送长度）_981) -> Out05_Handoff（输出交接与软件复位）/7(len1（电机发送长度）_992)
  Out04_Command（电机及油泵指令）/1(Tx1（电机九字节指令）_980) -> Out05_Handoff（输出交接与软件复位）/6(tx1（电机指令帧）_991)
  Out02_Timing（阀门与点火时序）/2(PortD（D口三路输出电平）_777) -> Out05_Handoff（输出交接与软件复位）/3(portD（D口三路电平）_988)
  Out02_Timing（阀门与点火时序）/1(PortE（E口三路输出电平）_775) -> Out05_Handoff（输出交接与软件复位）/2(portE（E口三路电平）_987)
  [BO_Control] -> Out05_Handoff（输出交接与软件复位）/1(Control（执行控制总线）_986)  "BO_Control（执行控制）"
  [BO_Send] -> Out04_Command（电机及油泵指令）/1(Send（外设命令总线）_867)  "BO_Send（回传命令）"
  [BO_Seconds] -> Out04_Command（电机及油泵指令）/2(Seconds（当前秒数）_868)  "BO_Seconds（当前时间）"
  [BO_Control] -> Out02_Timing（阀门与点火时序）/1(Control（执行控制总线）_682)  "BO_Control（执行控制）"
  Outputs（拆出原有八项输出）/1 -> PortE（E口三路电平）/1  "<portE>"
  Outputs（拆出原有八项输出）/2 -> PortD（D口三路电平）/1  "<portD>"
  Outputs（拆出原有八项输出）/3 -> Tx4（上位机回传帧）/1  "<tx4>"
  Outputs（拆出原有八项输出）/4 -> Length4（回传发送长度）/1  "<len4>"
  Outputs（拆出原有八项输出）/5 -> Tx1（电机指令帧）/1  "<tx1>"
  Outputs（拆出原有八项输出）/6 -> Length1（电机发送长度）/1  "<len1>"
  Outputs（拆出原有八项输出）/7 -> Tx2（油泵指令帧）/1  "<tx2>"
  Outputs（拆出原有八项输出）/8 -> Length2（油泵发送长度）/1  "<len2>"
  Out03_Telemetry（上位机回传组帧）/2(Length4（回传发送长度）_221) -> Out05_Handoff（输出交接与软件复位）/5(len4（上位机回传长度）_990)
  Out03_Telemetry（上位机回传组帧）/1(Tx4（上位机三十字节回传帧）_216) -> Out05_Handoff（输出交接与软件复位）/4(tx4（上位机回传帧）_989)
  [BO_Seconds] -> Out03_Telemetry（上位机回传组帧）/3(Seconds（当前秒数）_116)  "BO_Seconds（当前时间）"
  Out01_Pump（泵反馈解析与滤波）/1(Speed（反馈转速）_681) -> Out03_Telemetry（上位机回传组帧）/2(Pump（滤波后的油泵转速）_115)
  [BO_Send] -> Out03_Telemetry（上位机回传组帧）/1(Send（回传与外设命令总线）_114)  "BO_Send（回传命令）"
  PumpCount（油泵有效字节数）/1 -> Out01_Pump（泵反馈解析与滤波）/2(Count（有效字节数）_556)  "PumpCount（有效字节数）"
  PumpRx（油泵反馈字节）/1 -> Out01_Pump（泵反馈解析与滤波）/1(Rx（串口接收字节）_555)  "PumpRx（油泵反馈字节）"

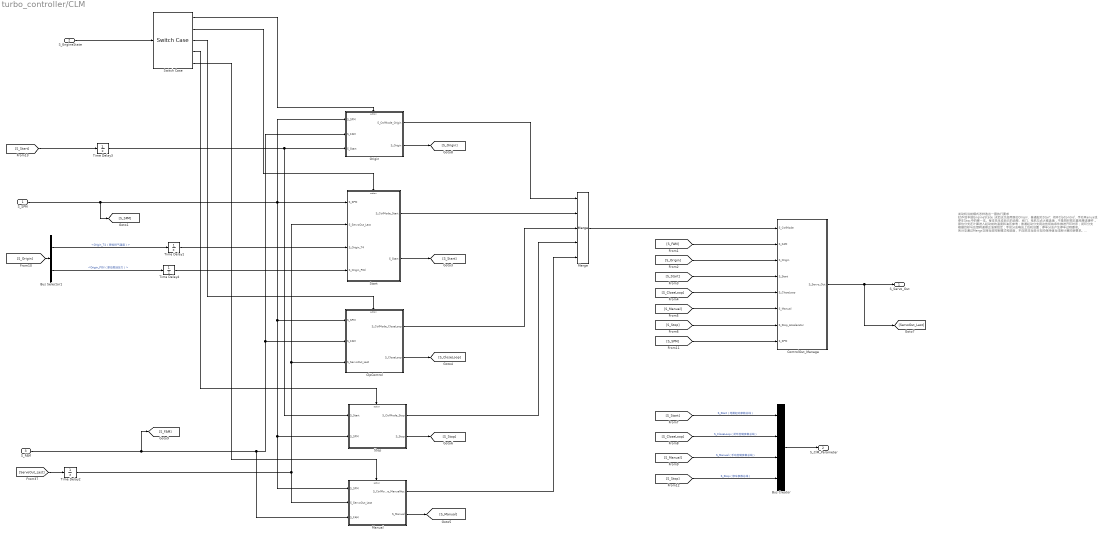
== system turbo_controller/CLM ==
  note: 发动机当前模式怎样选出一套执行要求
      |
      | ESM给本层EngineState，决定这次启用原位Origin、普通起动Start、闭环ClpControl、手动Manual或
      | 停车Stop中的哪一支。每支先生成自己的油泵、阀门、电机与点火候选值，不是同时把五套结果送硬件
      | 。
      |
      | 原位分支还计算进入起动前的温度和油压参考；普通起动分支用这些初始条件推进开环时序；闭环分支
      | 根据目标与反馈转速修正油泵给定；手动分支响应上位机设置；停车分支产生停车过程要求。
      | 各分支通过Merge交接当前控制模式和进度，不应把非当前分支的保持值当成刚计算的新要求。
      |
      | ControlOut_Manage最后统一仲裁：油泵给定按模式选择并限幅，阀门/电机/点火等字段按对应模式选
      | 择。结果组成S_Servo_Out，送ControlOut再到BoardOutput生成物理电平和串口帧。
      |
      | 上一周期执行输出和原位参考通过延迟回到本层，供增量PI、手动保持和初始值锁存使用。当前输入与
      | 上一周期值是不同用途，删掉记忆反馈会改变算法。当前只保留普通Start，已没有AirStart/BWStart
      | 分支。
  S_SPM : Inport
      settings: AttributesFormatString=S_SPM（通信及传感器信息总线）
  S_EngineState : Inport  Port=2
      settings: AttributesFormatString=S_EngineState（发动机状态）
  S_FAM : Inport  Port=3
      settings: AttributesFormatString=S_FAM（故障标志总线）
  Bus Creator : BusCreator  Inputs=4
      settings: AttributesFormatString=Bus Creator（总线创建器）
  Bus Selector1 : BusSelector  OutputSignals=Origin_T4（原位排气温度）,Origin_POil（原位燃油压力）
      settings: AttributesFormatString=Bus Selector1（总线选择器1）
  ClpControl : Subsystem  Description=|  TreatAsAtomicUnit=on
      | 闭环怎样根据转速偏差调整油泵
      | 
      | 本模块在发动机闭环模式运行。输入S_SPM含目标转速、实际滤波转速和入口压力，S_FAM提供转速故障标志，上一执行总线提供上次油泵给定。这里的Accelerator是油泵给定控制量，不能直接当作角度或占空比。
      | 
      | 先由Aim__Parameter_Calculate限制目标变化、给出油泵上下限和Kp/Ki。目标进入闭环时从当前转速逐步移动，避免突然把一个远离实际值的装订量全部加到控制律。
      | CtrlLaw计算目标减反馈的误差，用增量PI算本周期油泵变化量；小误差保持旧值，变化量按入口压力缩放并限幅。
      | 
      | Fault_Process再看转速传感器故障：短时故障可冻结上次给定，锁存故障时改用装订转速/高度插值的备用给定，并限制变化步长。正常时采用PI结果。
      | 最终候选给定和Kp/Ki、目标、给定上下限等参数组成闭环输出总线，交ControlOut_Manage再做模式统一选择；不会直接在这里发送油泵串口命令。
      settings: AttributesFormatString=ClpControl（闭环调速）
  ControlOut_Manage : Subsystem  Description=|  TreatAsAtomicUnit=on
      | 把当前模式的候选值合成统一执行总线
      | 
      | 前面的Origin、Start、ClpControl、Manual、Stop分别算出了候选控制。本层接收这些结果和当前控制模式，不让五套候选同时驱动硬件。
      | 
      | Accelerator_Manage负责油泵：按模式选出给定，闭环和手动分别受各自上下限约束；若复位恢复工作标志成立，采用恢复油泵值覆盖普通选择。
      | SWO_Manage负责主副阀、电机、点火与引气等字段：根据模式执行对应动作分支，再用Merge合成唯一结果。
      | 
      | 最后Bus Creator按固定字段组成S_Servo_Out，包含油泵给定、各执行机构周期/开启计数/使能，以及点火等开关要求。ServoCtrlFlag记录油泵究竟来自正常分支还是上下限分支，供诊断使用。
      | 
      | 输出交根层ControlOut整理端口，再由BoardOutput把周期计数变成电平、把给定变成串口帧。本模块完成的是控制量仲裁，尚未执行实际GPIO/UART动作。
      settings: AttributesFormatString=ControlOut_Manage（控制输出管理）
  Manual : Subsystem  Description=|  TreatAsAtomicUnit=on
      | 接收手动命令，分别保持各执行器的设定
      | 
      | 只有运行模式选到Manual时，本分支的结果才参与最终输出。它把“新一帧有效、命令编号、命令数据”送往各执行器，避免一条泵命令同时改动阀门或点火器。
      | 
      | 主油阀、副油阀分别设置开通比例；起动电机设置0～100的开通计数；点火器和引气阀把数据是否大于等于1变成开关。没有对应的新命令时，各通道保留自己的原设定，而不是全部清零。
      | 
      | 油泵另有直接给定和加减两条途径，并受转速保护及范围限制。手动输出仍要经过ControlOut_Manage、ControlOut和板级输出，才形成UART字节或GPIO电平；手动设定并不等于硬件已执行成功。
      settings: AttributesFormatString=Manual（手动）
  Merge : Merge  Inputs=5
      settings: AttributesFormatString=Merge（条件分支输出合并）
  Origin : Subsystem  Description=|  TreatAsAtomicUnit=on
      | 发动机初始模式：关闭常规驱动，准备起动参考值
      | 
      | 此分支在Origin模式下运行，给主、副油阀和电机准备默认周期与关闭设定。它还把当前T4和前4拍T4求平均，把当前油压和前4拍油压求平均，作为起动前参考排温和参考油压。后续普通起动实际采用油压参考，保持后的排温参考当前接终止端。
      | 
      | 公式：参考值=(本拍+前1拍+前2拍+前3拍+前4拍)/5。单拍毛刺只占五分之一，有利于后续判断油压是否相对起动前上升。
      | 
      | 内部保留Cool_Control冷却顺序，但当前接入它的Flag_Cool是常量0，正常连接下不会发起该冷却过程。不要仅因看到冷却控制图就认为初始模式一定会开电机吹冷。输出分别送模式选择和Start的参考值保持路径。
      settings: AttributesFormatString=Origin（原位）
  Start : Subsystem  Description=|  TreatAsAtomicUnit=on
      | 普通起动：先记住起动前状态，再按阶段控制供油与电机
      | 
      | 进入Start分支时，先保持起动前排温、油压；当前真正送入起动图的是油压参考，排温参考输出接终止端。参数支路根据滤波油压及历史参数准备初始电机开度、供油曲线和时间参数。
      | 
      | Start_OpenLoop随后按A～F推进：准备、拖转、建立油压与供油、继续加速、退出起动电机、转入闭环。各阶段会同时修改油泵给定、主副油阀、电机和点火许可，并检查转速、油压与超时。
      | 
      | 本系统只保留普通起动。阶段完成或异常的标志送回发动机状态管理，驱动量则经过统一输出管理后执行；内部某个阶段标志不是硬件执行成功的回执。
      settings: AttributesFormatString=Start（地面起动）
  Stop : Subsystem  Description=|  TreatAsAtomicUnit=on
      | 停车模式：停止供油并按条件处理尾部拖转
      | 
      | 停车命令进入本分支后，常规油泵给定转为停车值，Stop_Control结合命令、当前转速、排温及运行状态决定阀门和电机动作。
      | 
      | StopZero用于快速完成停车路径；普通停车保留等待、关闭油路及高温低转速时的电机拖转判断。Stop_Finish输出送发动机状态管理，控制数值和使能送统一输出管理。
      | 
      | “停车完成”是控制逻辑的完成标志，不是由此模块直接证明轴已完全静止。实际转速仍由独立测速链路采集。
      settings: AttributesFormatString=Stop（停车）
  Switch Case : SwitchCase  CaseConditions={PG_ES_Origin,PG_ES_EngStart,PG_ES_Clp,PG_ES_Stop,PG_ES_Manual}  ShowDefaultCase=off
      settings: AttributesFormatString=Switch Case（开关选择分支情况）
  Time Delay{1..4} (4 alike) : UnitDelay  SampleTime=-1  HasFrameUpgradeWarning=on
      Time Delay1 settings: AttributesFormatString=Time Delay1（时间延迟1）
      Time Delay2 settings: AttributesFormatString=Time Delay2（时间延迟2）
      Time Delay3 settings: AttributesFormatString=Time Delay3（时间延迟3）
      Time Delay4 settings: AttributesFormatString=Time Delay4（时间延迟4）
  S_Servo_Out : Outport
      settings: AttributesFormatString=S_Servo_Out（伺服输出）
  S_ClM_Parameter : Outport  Port=2
      settings: AttributesFormatString=S_ClM_Parameter（控制规律管理模块参数）
  wires:
  S_FAM/1 -> Origin/2(S_FAM), ClpControl/2(S_FAM), Manual/3(S_FAM), [S_FAM]
  [ServoOut_Last] -> Time Delay2/1
  S_SPM/1 -> Origin/1(S_SPM), Start/1(S_SPM), Manual/1(S_SPM), Stop/2(S_SPM), ClpControl/1(S_SPM), [S_SPM]
  Bus Creator/1 -> S_ClM_Parameter/1
  Start/2(S_Start) -> [S_Start]
  [S_FAM] -> ControlOut_Manage/2(S_FAM)
  ClpControl/2(S_CloseLoop) -> [S_CloseLoop]
  Stop/2(S_Stop) -> [S_Stop]
  Manual/2(S_Manual) -> [S_Manual]
  [S_Stop] -> ControlOut_Manage/7(S_Stop_Accelerator)
  [S_Origin] -> ControlOut_Manage/3(S_Origin)
  [S_Start] -> ControlOut_Manage/4(S_Start)
  [S_CloseLoop] -> ControlOut_Manage/5(S_CloseLoop)
  [S_Manual] -> ControlOut_Manage/6(S_Manual)
  [S_Manual] -> Bus Creator/3  "S_Manual（手动控制参数总线）"
  [S_CloseLoop] -> Bus Creator/2  "S_CloseLoop（闭环控制参数总线）"
  [S_Start] -> Bus Creator/1  "S_Start（地面起动参数总线）"
  ControlOut_Manage/1(S_Servo_Out) -> [ServoOut_Last], S_Servo_Out/1
  Origin/2(S_Origin) -> [S_Origin]
  [S_SPM] -> ControlOut_Manage/8(S_SPM)
  [S_Origin] -> Bus Selector1/1
  [S_Stop] -> Bus Creator/4  "S_Stop（停车参数总线）"
  Bus Selector1/1 -> Time Delay1/1  "<Origin_T4（原位排气温度）>"
  Time Delay1/1 -> Start/3(S_Origin_T4)
  Time Delay2/1 -> ClpControl/3(S_ServoOut_Last), Start/2(S_ServoOut_Last), Manual/2(S_ServoOut_Last)
  [S_Start] -> Time Delay3/1
  Bus Selector1/2 -> Time Delay4/1  "<Origin_POil（原位燃油压力）>"
  Time Delay4/1 -> Start/4(S_Origin_POil)
  Time Delay3/1 -> Stop/1(S_Start), Origin/3(S_Start)
  Manual/1(S_CtrlMode_ManualAcc) -> Merge/5
  Switch Case/5 -> Manual/Action
  Stop/1(S_CtrlMode_Stop) -> Merge/4
  Switch Case/4 -> Stop/Action
  ClpControl/1(S_CtrlMode_CloseLoop) -> Merge/3
  Start/1(S_CtrlMode_Start) -> Merge/2
  Switch Case/2 -> Start/Action
  Origin/1(S_CtrlMode_Origin) -> Merge/1
  Switch Case/1 -> Origin/Action
  Switch Case/3 -> ClpControl/Action
  S_EngineState/1 -> Switch Case/1
  Merge/1 -> ControlOut_Manage/1(S_CtrlMode)

== system turbo_controller/COMMRead_ISM ==
  note: 把通信输入和板载采样整理成控制器可用的数据
      |
      | 这是输入侧的汇合处。CMMRead负责解释上位机命令、目标转速、环境和飞行信息；ISM负责把板载ADC
      | 与测速数据标定、筛选、滤波，输出传感器总线。两类来源分开保留，名称相近也不代表同一测量。
      |
      | 例如ADC供电电压用于监视与回传，而通信中的V_Power来自上位机字段；排温经过标定、低通后进入起
      | 动及告警。温度修正转速另用于记录和回传，不应与闭环采用的Nc_Filter混用。
      |
      | 内部还有复位记录解码接口，但当前恢复使能接常量false，外部FRAM有效标志未实际投入这条恢复选
      | 择。Dynamic_Cal虽然计算总温总压，送到ISM转速修正接口的T1t当前仍为288.15 K常量。注释按现有
      | 连接说明，不能把预留算法当作已投入功能。
  S_Flag_rx_suc : Inport
      settings: AttributesFormatString=S_Flag_rx_suc（四号串口指令帧有效标志）
  S_PF_MyUsart2_Rxdata : Inport  Port=2
      settings: AttributesFormatString=S_PF_MyUsart2_Rxdata（本通道通用同步异步串行通信接口2接收数据）
  S_Flag_ECUReset : Inport  Port=3
      settings: AttributesFormatString=S_Flag_ECUReset（复位恢复标志）
  S_ECUReset_Information : Inport  Port=4
      settings: AttributesFormatString=S_ECUReset_Information（铁电存储器中的复位恢复记录）
  S_MySet_Rxdata : Inport  Port=5
      settings: AttributesFormatString=S_MySet_Rxdata（板端配置缓冲区）
  S_Nc : Inport  Port=6
      settings: AttributesFormatString=S_Nc（发动机反馈转速（转每分））
  S_T4 : Inport  Port=7
      settings: AttributesFormatString=S_T4（排温ADC采样码（未换算℃））
  S_Vpower : Inport  Port=8
      settings: AttributesFormatString=S_Vpower（板端换算电源电压）
  S_Tecu : Inport  Port=9
      settings: AttributesFormatString=S_Tecu（处理器温度ADC采样码）
  S_SWI_Firework : Inport  Port=10
      settings: AttributesFormatString=S_SWI_Firework（点火器报警反馈（低有效））
  S_SWI_EValve : Inport  Port=11
      settings: AttributesFormatString=S_SWI_EValve（主油阀反馈（低有效））
  S_SWI_Eblast : Inport  Port=12
      settings: AttributesFormatString=S_SWI_Eblast（副油阀反馈（低有效））
  S_SWI_ValveErr : Inport  Port=13
      settings: AttributesFormatString=S_SWI_ValveErr（任一路阀报警（低有效））
  S_EngineState : Inport  Port=14
      settings: AttributesFormatString=S_EngineState（发动机状态）
  S_SWI_BleedAir : Inport  Port=15
      settings: AttributesFormatString=S_SWI_BleedAir（引气阀反馈（低有效））
  S_POil : Inport  Port=16
      settings: AttributesFormatString=S_POil（油压输入：模型需采样码／板端传电压）
  S_T0 : Inport  Port=17
      settings: AttributesFormatString=S_T0（板端总温编码（℃＋80））
  Bus Creator1 : BusCreator  Inputs=19
      settings: AttributesFormatString=Bus Creator1（总线创建器1）
  Bus Creator2 : BusCreator  Inputs=2
      settings: AttributesFormatString=Bus Creator2（总线创建器2）
  CMMRead : Subsystem  Description=|  Priority=0  TreatAsAtomicUnit=on
      | 把已校验的上位机帧解释为命令和运行设定
      | 
      | 输入是接收层保留下来的帧、接收成功标志和当前发动机模式。先由Instr_Analyse识别命令，再由SpeedLoad_Analyse确定本次目标转速，同时解析高度、空速、环境温度、电压等协议字段。
      | 
      | 一帧数据并不是全部都用于当前控制。命令类型决定哪些字段有效；没有新有效信息时，需要保持的设定沿用历史值。闭环目标、起动默认目标和停车目标有各自的选择路径。
      | 
      | 本层负责“字节是什么意思”；校验与收帧在BoardInput内完成，实际驱动在CLM和BoardOutput完成。输出的通信电压、环境信息也不能与ADC测得的同名量混为一谈。
      settings: AttributesFormatString=CMMRead（通信读取）
  Constant : Constant  Value=288.15
      settings: AttributesFormatString=Constant（常量）
  Constant13 : Constant  Value=false  SampleTime=-1
      settings: AttributesFormatString=Constant13（常量13）
  Data Type Conversion : DataTypeConversion  OutDataTypeStr=single  SaturateOnIntegerOverflow=off  RndMeth=Floor
      settings: AttributesFormatString=Data Type Conversion（数据类型转换）
  Data Type Conversion1 : DataTypeConversion  OutDataTypeStr=single  SaturateOnIntegerOverflow=off  RndMeth=Floor
      settings: AttributesFormatString=Data Type Conversion1（数据类型转换1）
  ECUReset_Information_Read : Subsystem  Description=|  TreatAsAtomicUnit=on
      | 从恢复字节中取回泵给定、目标转速和原运行模式
      | 
      | 输入是FRAM恢复信息数组与有效标志。泵给定用两个字节高位在前合成，目标转速用三个字节合成；发动机模式由指定字节直接取出。
      | 
      | 有效恢复不只看数组里有没有非零值，还要经过目标转速30000～89000的范围判断并与恢复标志组合。输出分别供目标选择、恢复期间泵输出及模式判断使用。
      | 
      | 当前COMMRead_ISM把恢复标志接为false，尽管这些解码支路仍在，正常运行不会采用恢复记录。不要把“可以解码”解释为“复位后已经按该值恢复运行”。
      settings: AttributesFormatString=ECUReset_Information_Read（控制器复位信息读取）
  ISM : Subsystem  Description=|  TreatAsAtomicUnit=on
      | 把测量输入整理成控制算法能取用的Sensor总线
      | 
      | 本层接收的输入并不全是同一类数据：排温、油压和芯片温度仍有原始计数；电源电压已经在BoardInput换算成V；T0则是加80后的温度编码。先认清这一点，才能理解为什么各路处理不同。
      | 
      | 排温走Calibrating_T4三级查表，再走AnalogFilter_T4，得到平滑的T4_Filter。标定后的排温还分一路到Subsystem2，以930 ℃上限生成排温超限标志；这一路标志当前没有查到下游取用。
      | 油压走Calibrating_Poil，将计数换为电压、再换为压力，然后AnalogFilter_Poil平滑，得到POil_Filter。
      | 芯片温度走Calibrating_Tecu，先换电压，再按0.76 V和25 ℃参考关系计算Tecu。
      | 总温走Calibrating_T0，减去80并限制在-70～175 ℃；再与原位滤波转速送入HuanSuanN，计算温度修正转速。
      | 电源电压Vpower已经是V，本层直接转交，不再做独立低通滤波。
      | 
      | 转速来自捕获/电机链路，不来自ADC。它一方面进入AnalogFilter_Nc作异常检查和滤波；另一方面进入Origin_Nc_Filter，形成原位转速，供总温修正使用。
      | 点火、阀门等数字反馈按字段转交。
      | 
      | 最后Bus Creator3按名称把上述结果装进Sensor总线，再由父级与COMM总线合成S_SPM。总线只是打包，不再次计算数值。CLM、MAM、SaveData和SendData分别取所需字段，因此标定值、滤波值和故障标志要分开理解。
      settings: AttributesFormatString=ISM（输入信号管理模块）
  MySet_Rxdatan_Read : Subsystem  Description=|  TreatAsAtomicUnit=on
      | 从配置数据里取出软件版本的三个部分
      | 
      | 按协议位置分别提取高、中、低版本字段，输出Soft_H、Soft_M、Soft_L。这里不做ADC采样、不比较版本新旧，也不把三个字段合成转速或压力。
      | 
      | 这三项后续参与状态记录或回传，使上位机能识别当前控制软件版本。各字节的含义由配置协议约定；例如高、中、低分别是1、2、3时，它们仍是三个独立字段，并非自动成为十进制123。
      settings: AttributesFormatString=MySet_Rxdatan_Read（本通道设置接收数据读取）
  Terminator4 : Terminator
      settings: AttributesFormatString=Terminator4（终止未使用信号4）
  S_SPM : Outport
      settings: AttributesFormatString=S_SPM（通信及传感器信息总线）
  wires:
  Bus Creator1/1 -> Bus Creator2/1  "COMM（通信信息总线）"
  S_T4/1 -> ISM/2(S_T4)
  S_Vpower/1 -> ISM/3(S_Vpower)
  S_Nc/1 -> ISM/5(S_Nc)
  S_SWI_Firework/1 -> ISM/6(S_SWI_Firework)
  S_SWI_EValve/1 -> ISM/7(S_SWI_EValve)
  S_SWI_Eblast/1 -> ISM/8(S_SWI_Eblast)
  ISM/1(S_Sensor) -> Bus Creator2/2  "Sensor（传感器信息总线）"
  Constant13/1 -> ECUReset_Information_Read/1(S_Flag_ECUReset)
  ECUReset_Information_Read/2(S_ECUReset_Acclerator) -> Bus Creator1/2  "ECUReset_Acclerator（复位恢复油泵给定）"
  ECUReset_Information_Read/3(S_ECUReset_NcDem) -> Bus Creator1/3, [ECUReset_NcDem]  "ECUReset_NcDem（复位恢复目标转速）"
  ECUReset_Information_Read/4(S_ECUReset_EngineState) -> Bus Creator1/4  "ECUReset_EngineState（复位恢复发动机状态）"
  S_ECUReset_Information/1 -> ECUReset_Information_Read/2(S_ECUReset_Information)
  S_Tecu/1 -> ISM/4(S_Tecu)
  S_MySet_Rxdata/1 -> MySet_Rxdatan_Read/1(S_MySet_Rxdata)
  ECUReset_Information_Read/1(S_Flag_ECUReset_Use) -> [Flag_ECUReset_Use], Bus Creator1/1  "Flag_ECUReset_Use（复位恢复数据使用标志）"
  Constant/1 -> ISM/1(S_T1t_calc)
  S_Flag_rx_suc/1 -> CMMRead/1(S_Flag_rx_suc)
  S_PF_MyUsart2_Rxdata/1 -> CMMRead/2(S_PF_MyUsart2_Rxdata)
  S_Flag_ECUReset/1 -> Terminator4/1
  MySet_Rxdatan_Read/3(S_Soft_L) -> Bus Creator1/19  "Soft_L（软件版本低字节）"
  MySet_Rxdatan_Read/2(S_Soft_M) -> Bus Creator1/18  "Soft_M（软件版本中字节）"
  MySet_Rxdatan_Read/1(S_Soft_H) -> Bus Creator1/17  "Soft_H（软件版本高字节）"
  [Flag_ECUReset_Use] -> CMMRead/3(S_Flag_ECUReset_Use)
  [ECUReset_NcDem] -> CMMRead/4(S_ECUReset_NcDem)
  S_EngineState/1 -> [EngineState]
  [EngineState] -> ISM/10(S_EngineState)
  [EngineState] -> CMMRead/5(S_EngineState)
  CMMRead/1(S_Rx_suc) -> Bus Creator1/5  "Flag_rx_suc（接收成功标志）"
  CMMRead/2(S_Instr_XianShi) -> Bus Creator1/6  "Instr_XianShi（指令回显）"
  CMMRead/3(S_Instr_Out) -> Bus Creator1/7  "Instr（控制指令）"
  CMMRead/4(S_SpeedLoad) -> Bus Creator1/8  "SpeedLoad（装订转速）"
  CMMRead/5(T0_calc) -> Data Type Conversion/1
  CMMRead/8(H_GPRS) -> Bus Creator1/12  "H_Gprs（导航高度）"
  CMMRead/9(AirSpeed) -> Bus Creator1/13  "AirSpeed（飞行空速）"
  S_SWI_ValveErr/1 -> ISM/9(S_SWI_ValveErr)
  Data Type Conversion1/1 -> Bus Creator1/10  "T1t_calc（入口参考总温计算值）"
  Data Type Conversion/1 -> Bus Creator1/9  "T0_calc（入口总温计算值）"
  CMMRead/6(T1t_calc) -> Data Type Conversion1/1
  CMMRead/7(P1t_calc) -> Bus Creator1/11  "P1t_calc（入口总压计算值）"
  Bus Creator2/1 -> S_SPM/1
  CMMRead/10(S_COMM_Data6) -> Bus Creator1/14  "COMM_Data6（接收指令第六数据项）"
  S_SWI_BleedAir/1 -> ISM/11(S_SWI_BleedAir)
  CMMRead/11(H_Load) -> Bus Creator1/15  "H_Load（装订高度）"
  CMMRead/12(V_Power) -> Bus Creator1/16  "V_Power（电源电压）"
  S_POil/1 -> ISM/12(S_POil)
  S_T0/1 -> ISM/13(S_T0)
